simulink model "Architecture_261027_ver9"  (R2026b)
settings: Solver=FixedStepDiscrete  FixedStep=0.005
(part 2 of 2)

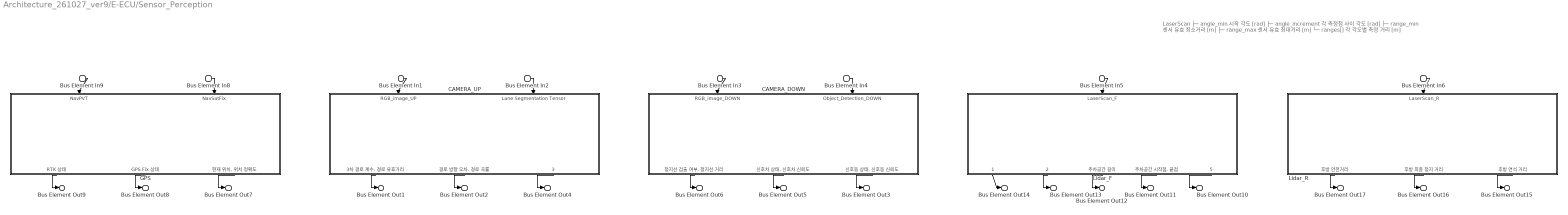
== system Architecture_261027_ver9/E-ECU/Sensor_Perception ==
  note: LaserScan
      | ├─ angle_min 시작 각도 [rad]
      | ├─ angle_increment 각 측정점 사이 각도 [rad]
      | ├─ range_min 센서 유효 최소거리 [m]
      | ├─ range_max 센서 유효 최대거리 [m]
      | └─ ranges[] 각 각도별 측정 거리 [m]
  Bus Element In1 : Inport  PortName=RGB_image_UP
  Bus Element In2 : Inport  Port=2  PortName=Lane Segmentation Tensor
  Bus Element In3 : Inport  Port=3  PortName=RGB_image_DOWN
  Bus Element In4 : Inport  Port=4  PortName=Object_Detection_DOWN
  Bus Element In5 : Inport  Port=5  PortName=LaserScan_F
  Bus Element In6 : Inport  Port=6  PortName=LaserScan_R
  Bus Element In9 : Inport  Port=7  PortName=NavPVT
  Bus Element In8 : Inport  Port=8  PortName=NavSatFix
  CAMERA_DOWN : Subsystem
      settings: PortSchema="{\"entries\":[{\"content\":{\"headerSize\":26,\"margin\":15,\"minimumSpacing\":25,\"sides\":[{\"content\":{},\"type\":\"ConnectorPlacement.EquallySpacedRectSide\",\"uuid\":\"3db2b88d-95e2-4692-a68d-7a6617ae29da\"},{\"content\":{\"side\":\"RIGHT\"},\"type\":\"ConnectorPlacement.EquallySpacedRectSide\",\"uuid\":\"d7a2bc47-76ea-49a7-91d2-0b0182d23db2\"},{\"content\":{\"connectorIds\":[\"In1\",\"In2\"],\"side\":\"TOP\"},\"type\":\"ConnectorPlacement.EquallySpacedRectSide\",\"uuid\":\"f0af930f-0cf6-4b9c-8a26-23e4e388c29c\"},{\"content\":{\"connectorIds\":[\"Out1\",\"Out2\",\"Out3\"],\"side\":\"BOTTOM\"},\"type\":\"ConnectorPlacement.EquallySpacedRectSide\",\"uuid\":\"67596a2e-158a-411e-8daf-83dd5bf86ad3\"}]},\"type\":\"ConnectorPlacement.EquallySpacedConnector\",\"uuid\":\"d65d877a-ca9e-4f5a-ba0a-bbaf7f04c4f0\"}],\"packageUris\":[\"http://schema.mathworks.com/mf0/Connector/R2020b\"],\"version\":\"1.0\"}"
  CAMERA_UP : Subsystem
      settings: PortSchema="{\"entries\":[{\"content\":{\"headerSize\":26,\"margin\":15,\"minimumSpacing\":25,\"sides\":[{\"content\":{},\"type\":\"ConnectorPlacement.EquallySpacedRectSide\",\"uuid\":\"3db2b88d-95e2-4692-a68d-7a6617ae29da\"},{\"content\":{\"side\":\"RIGHT\"},\"type\":\"ConnectorPlacement.EquallySpacedRectSide\",\"uuid\":\"d7a2bc47-76ea-49a7-91d2-0b0182d23db2\"},{\"content\":{\"connectorIds\":[\"In1\",\"In2\"],\"side\":\"TOP\"},\"type\":\"ConnectorPlacement.EquallySpacedRectSide\",\"uuid\":\"f0af930f-0cf6-4b9c-8a26-23e4e388c29c\"},{\"content\":{\"connectorIds\":[\"Out1\",\"Out2\",\"Out3\"],\"side\":\"BOTTOM\"},\"type\":\"ConnectorPlacement.EquallySpacedRectSide\",\"uuid\":\"de9f83c0-76b7-4878-914e-e95a158d2e20\"}]},\"type\":\"ConnectorPlacement.EquallySpacedConnector\",\"uuid\":\"d65d877a-ca9e-4f5a-ba0a-bbaf7f04c4f0\"}],\"packageUris\":[\"http://schema.mathworks.com/mf0/Connector/R2020b\"],\"version\":\"1.0\"}"
  GPS : Subsystem
      settings: PortSchema="{\"entries\":[{\"content\":{\"headerSize\":26,\"margin\":15,\"minimumSpacing\":25,\"sides\":[{\"content\":{},\"type\":\"ConnectorPlacement.EquallySpacedRectSide\",\"uuid\":\"3db2b88d-95e2-4692-a68d-7a6617ae29da\"},{\"content\":{\"side\":\"RIGHT\"},\"type\":\"ConnectorPlacement.EquallySpacedRectSide\",\"uuid\":\"d7a2bc47-76ea-49a7-91d2-0b0182d23db2\"},{\"content\":{\"connectorIds\":[\"In2\",\"In1\"],\"side\":\"TOP\"},\"type\":\"ConnectorPlacement.EquallySpacedRectSide\",\"uuid\":\"f0af930f-0cf6-4b9c-8a26-23e4e388c29c\"},{\"content\":{\"connectorIds\":[\"Out1\",\"Out2\",\"Out3\"],\"side\":\"BOTTOM\"},\"type\":\"ConnectorPlacement.EquallySpacedRectSide\",\"uuid\":\"c8f4bbcc-ac0b-4106-aebd-72f0ecd21f1b\"}]},\"type\":\"ConnectorPlacement.EquallySpacedConnector\",\"uuid\":\"d65d877a-ca9e-4f5a-ba0a-bbaf7f04c4f0\"}],\"packageUris\":[\"http://schema.mathworks.com/mf0/Connector/R2020b\"],\"version\":\"1.0\"}"
  Lidar_F : Subsystem
      settings: PortSchema="{\"entries\":[{\"content\":{\"headerSize\":26,\"margin\":15,\"minimumSpacing\":25,\"sides\":[{\"content\":{},\"type\":\"ConnectorPlacement.EquallySpacedRectSide\",\"uuid\":\"3db2b88d-95e2-4692-a68d-7a6617ae29da\"},{\"content\":{\"side\":\"RIGHT\"},\"type\":\"ConnectorPlacement.EquallySpacedRectSide\",\"uuid\":\"d7a2bc47-76ea-49a7-91d2-0b0182d23db2\"},{\"content\":{\"connectorIds\":[\"In1\"],\"side\":\"TOP\"},\"type\":\"ConnectorPlacement.EquallySpacedRectSide\",\"uuid\":\"f0af930f-0cf6-4b9c-8a26-23e4e388c29c\"},{\"content\":{\"connectorIds\":[\"Out1\",\"Out2\",\"Out3\",\"Out4\",\"Out5\"],\"side\":\"BOTTOM\"},\"type\":\"ConnectorPlacement.EquallySpacedRectSide\",\"uuid\":\"cd59c8ad-aa31-4ab1-b799-627b51476627\"}]},\"type\":\"ConnectorPlacement.EquallySpacedConnector\",\"uuid\":\"d65d877a-ca9e-4f5a-ba0a-bbaf7f04c4f0\"}],\"packageUris\":[\"http://schema.mathworks.com/mf0/Connector/R2020b\"],\"version\":\"1.0\"}"
  Lidar_R : Subsystem
      settings: PortSchema="{\"entries\":[{\"content\":{\"headerSize\":26,\"margin\":15,\"minimumSpacing\":25,\"sides\":[{\"content\":{},\"type\":\"ConnectorPlacement.EquallySpacedRectSide\",\"uuid\":\"3db2b88d-95e2-4692-a68d-7a6617ae29da\"},{\"content\":{\"side\":\"RIGHT\"},\"type\":\"ConnectorPlacement.EquallySpacedRectSide\",\"uuid\":\"d7a2bc47-76ea-49a7-91d2-0b0182d23db2\"},{\"content\":{\"connectorIds\":[\"In1\"],\"side\":\"TOP\"},\"type\":\"ConnectorPlacement.EquallySpacedRectSide\",\"uuid\":\"f0af930f-0cf6-4b9c-8a26-23e4e388c29c\"},{\"content\":{\"connectorIds\":[\"Out1\",\"Out2\",\"Out3\"],\"side\":\"BOTTOM\"},\"type\":\"ConnectorPlacement.EquallySpacedRectSide\",\"uuid\":\"d0e0971b-ab0f-4249-9f75-3116b1a494cb\"}]},\"type\":\"ConnectorPlacement.EquallySpacedConnector\",\"uuid\":\"d65d877a-ca9e-4f5a-ba0a-bbaf7f04c4f0\"}],\"packageUris\":[\"http://schema.mathworks.com/mf0/Connector/R2020b\"],\"version\":\"1.0\"}"
  Bus Element Out17 : Outport  PortName=후방 안전거리
  Bus Element Out16 : Outport  Port=2  PortName=후방 최종 정지 거리
  Bus Element Out15 : Outport  Port=3  PortName=후방 연석 거리
  Bus Element Out14 : Outport  Port=4  PortName=전방 주행 경로 내 장애물 여부
  Bus Element Out1 : Outport  Port=5  PortName=3차 경로 계수, 경로 유효거리
  Bus Element Out2 : Outport  Port=6  PortName=경로 방향 오차, 경로 곡률
  Bus Element Out4 : Outport  Port=7  PortName=차선/경로 유효 여부, 신뢰도, 차량 횡방향 오차
  Bus Element Out13 : Outport  Port=8  PortName=전방 장애물 거리, 폭, 좌우 위치
  Bus Element Out12 : Outport  Port=9  PortName=주차공간 길이
  Bus Element Out11 : Outport  Port=10  PortName=주차공간 시작점, 끝점
  Bus Element Out10 : Outport  Port=11  PortName=전방 연석 검출 여부, 측면 연석 거리
  Bus Element Out9 : Outport  Port=12  PortName=RTK 상태
  Bus Element Out8 : Outport  Port=13  PortName=GPS Fix 상태
  Bus Element Out5 : Outport  Port=14  PortName=신호차 상태, 신호차 신뢰도
  Bus Element Out7 : Outport  Port=15  PortName=현재 위치, 위치 정확도
  Bus Element Out6 : Outport  Port=16  PortName=정지선 검출 여부, 정지선 거리
  Bus Element Out3 : Outport  Port=17  PortName=신호등 상태, 신호등 신뢰도
  wires:
  CAMERA_DOWN/2("신호차 상태, 신호차 신뢰도") -> Bus Element Out5/1
  CAMERA_DOWN/1("정지선 검출 여부, 정지선 거리") -> Bus Element Out6/1
  CAMERA_DOWN/3("신호등 상태, 신호등 신뢰도") -> Bus Element Out3/1
  GPS/1(RTK 상태) -> Bus Element Out9/1
  GPS/2(GPS Fix 상태) -> Bus Element Out8/1
  GPS/3("현재 위치, 위치 정확도") -> Bus Element Out7/1
  Lidar_F/1(전방 주행 경로 내 장애물 여부) -> Bus Element Out14/1
  Lidar_F/2("전방 장애물 거리, 폭, 좌우 위치") -> Bus Element Out13/1
  Lidar_F/3(주차공간 길이) -> Bus Element Out12/1
  Lidar_F/4("주차공간 시작점, 끝점") -> Bus Element Out11/1
  Lidar_F/5("전방 연석 검출 여부, 측면 연석 거리") -> Bus Element Out10/1
  Lidar_R/3(후방 연석 거리) -> Bus Element Out15/1
  Lidar_R/2(후방 최종 정지 거리) -> Bus Element Out16/1
  Lidar_R/1(후방 안전거리) -> Bus Element Out17/1
  Bus Element In8/1 -> GPS/1("NavSatFix ")
  Bus Element In9/1 -> GPS/2(NavPVT)
  Bus Element In1/1 -> CAMERA_UP/1(RGB_image_UP)
  Bus Element In3/1 -> CAMERA_DOWN/1(RGB_image_DOWN)
  Bus Element In4/1 -> CAMERA_DOWN/2(Object_Detection_DOWN)
  Bus Element In6/1 -> Lidar_R/1(LaserScan_R)
  Bus Element In5/1 -> Lidar_F/1(LaserScan_F)
  Bus Element In2/1 -> CAMERA_UP/2(Lane Segmentation Tensor)
  CAMERA_UP/1("3차 경로 계수, 경로 유효거리") -> Bus Element Out1/1
  CAMERA_UP/2("경로 방향 오차, 경로 곡률") -> Bus Element Out2/1
  CAMERA_UP/3("차선/경로 유효 여부, 신뢰도, 차량 횡방향 오차") -> Bus Element Out4/1

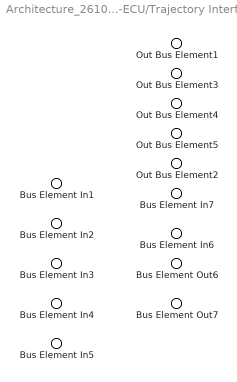
== system Architecture_261027_ver9/E-ECU/Trajectory Interface ==
  Bus Element In1 : Inport  PortName=GPS_Trajectory
  Bus Element In2 : Inport  Port=2  PortName=TParking_Trajectory
  Bus Element In3 : Inport  Port=3  PortName=ParallelParking_Trajectory
  Bus Element In4 : Inport  Port=4  PortName=Avoidance_Trajectory
  Bus Element In5 : Inport  Port=5  PortName=Camera_Trajectory
  Bus Element In7 : Inport  Port=6  PortName=Traffic_Stop_Request
  Bus Element In6 : Inport  Port=7  PortName=MRM_Stop_Request
  Out Bus Element1 : Outport  PortName=""
  Out Bus Element2 : Outport  Port=2  PortName=""
  Out Bus Element3 : Outport  Port=3  PortName=""
  Out Bus Element4 : Outport  Port=4  PortName=""
  Out Bus Element5 : Outport  Port=5  PortName=""
  Bus Element Out6 : Outport  Port=6  PortName=""
  Bus Element Out7 : Outport  Port=7  PortName=""

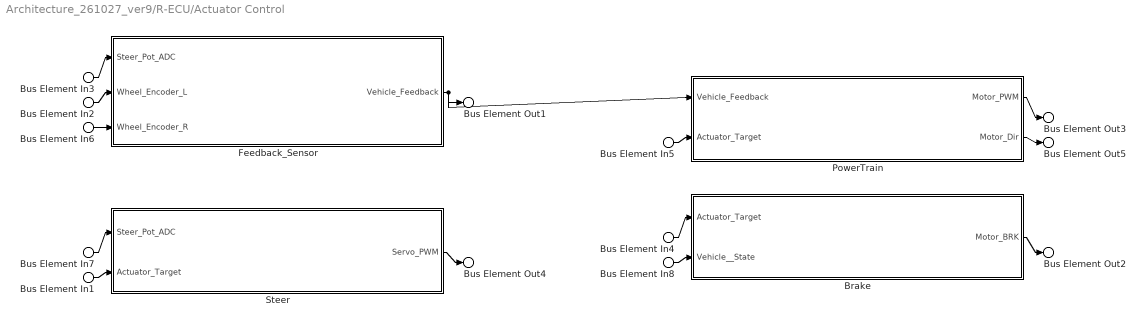
== system Architecture_261027_ver9/R-ECU/Actuator Control ==
  Bus Element In1 : Inport  PortName=Actuator_Target
  Bus Element In4 : Inport  PortName=Actuator_Target
  Bus Element In5 : Inport  PortName=Actuator_Target
  Bus Element In8 : Inport  Port=2  PortName=Vehicle__State
  Bus Element In2 : Inport  Port=3  PortName=Wheel_Encoder_L
  Bus Element In6 : Inport  Port=4  PortName=Wheel_Encoder_R
  Bus Element In3 : Inport  Port=5  PortName=Steer_Pot_ADC
  Bus Element In7 : Inport  Port=5  PortName=Steer_Pot_ADC
  Brake : Subsystem
      settings: PortSchema="{\"entries\":[{\"content\":{\"headerSize\":26,\"margin\":15,\"minimumSpacing\":25,\"sides\":[{\"content\":{\"connectorIds\":[\"In1\",\"In2\"]},\"type\":\"ConnectorPlacement.EquallySpacedRectSide\",\"uuid\":\"5be6b78a-1fb5-4892-a059-20486cb8da03\"},{\"content\":{\"connectorIds\":[\"Out1\"],\"side\":\"RIGHT\"},\"type\":\"ConnectorPlacement.EquallySpacedRectSide\",\"uuid\":\"6033bdc5-529e-4fd7-96df-de1a61a0c34f\"},{\"content\":{\"side\":\"TOP\"},\"type\":\"ConnectorPlacement.EquallySpacedRectSide\",\"uuid\":\"4d265f78-1951-4f58-a661-9dd8a9ad83fa\"}]},\"type\":\"ConnectorPlacement.EquallySpacedConnector\",\"uuid\":\"a5be31a5-398c-4cfa-a3f1-90989462f386\"}],\"packageUris\":[\"http://schema.mathworks.com/mf0/Connector/R2020b\"],\"version\":\"1.0\"}"
  Feedback_Sensor : Subsystem
      settings: PortSchema="{\"entries\":[{\"content\":{\"headerSize\":26,\"margin\":15,\"minimumSpacing\":25,\"sides\":[{\"content\":{\"connectorIds\":[\"In1\",\"In2\",\"In3\"]},\"type\":\"ConnectorPlacement.EquallySpacedRectSide\",\"uuid\":\"5be6b78a-1fb5-4892-a059-20486cb8da03\"},{\"content\":{\"connectorIds\":[\"Out1\"],\"side\":\"RIGHT\"},\"type\":\"ConnectorPlacement.EquallySpacedRectSide\",\"uuid\":\"6033bdc5-529e-4fd7-96df-de1a61a0c34f\"},{\"content\":{\"side\":\"TOP\"},\"type\":\"ConnectorPlacement.EquallySpacedRectSide\",\"uuid\":\"4d265f78-1951-4f58-a661-9dd8a9ad83fa\"}]},\"type\":\"ConnectorPlacement.EquallySpacedConnector\",\"uuid\":\"a5be31a5-398c-4cfa-a3f1-90989462f386\"}],\"packageUris\":[\"http://schema.mathworks.com/mf0/Connector/R2020b\"],\"version\":\"1.0\"}"
  PowerTrain : Subsystem
      settings: PortSchema="{\"entries\":[{\"content\":{\"headerSize\":26,\"margin\":15,\"minimumSpacing\":25,\"sides\":[{\"content\":{\"connectorIds\":[\"In1\",\"In2\"]},\"type\":\"ConnectorPlacement.EquallySpacedRectSide\",\"uuid\":\"5be6b78a-1fb5-4892-a059-20486cb8da03\"},{\"content\":{\"connectorIds\":[\"Out1\",\"Out2\"],\"side\":\"RIGHT\"},\"type\":\"ConnectorPlacement.EquallySpacedRectSide\",\"uuid\":\"6033bdc5-529e-4fd7-96df-de1a61a0c34f\"},{\"content\":{\"side\":\"TOP\"},\"type\":\"ConnectorPlacement.EquallySpacedRectSide\",\"uuid\":\"4d265f78-1951-4f58-a661-9dd8a9ad83fa\"}]},\"type\":\"ConnectorPlacement.EquallySpacedConnector\",\"uuid\":\"a5be31a5-398c-4cfa-a3f1-90989462f386\"}],\"packageUris\":[\"http://schema.mathworks.com/mf0/Connector/R2020b\"],\"version\":\"1.0\"}"
  Steer : Subsystem
      settings: PortSchema="{\"entries\":[{\"content\":{\"headerSize\":26,\"margin\":15,\"minimumSpacing\":25,\"sides\":[{\"content\":{\"connectorIds\":[\"In1\",\"In2\"]},\"type\":\"ConnectorPlacement.EquallySpacedRectSide\",\"uuid\":\"5be6b78a-1fb5-4892-a059-20486cb8da03\"},{\"content\":{\"connectorIds\":[\"Out1\"],\"side\":\"RIGHT\"},\"type\":\"ConnectorPlacement.EquallySpacedRectSide\",\"uuid\":\"6033bdc5-529e-4fd7-96df-de1a61a0c34f\"},{\"content\":{\"side\":\"TOP\"},\"type\":\"ConnectorPlacement.EquallySpacedRectSide\",\"uuid\":\"4d265f78-1951-4f58-a661-9dd8a9ad83fa\"}]},\"type\":\"ConnectorPlacement.EquallySpacedConnector\",\"uuid\":\"a5be31a5-398c-4cfa-a3f1-90989462f386\"}],\"packageUris\":[\"http://schema.mathworks.com/mf0/Connector/R2020b\"],\"version\":\"1.0\"}"
  Bus Element Out5 : Outport  PortName=Motor_DIR
  Bus Element Out1 : Outport  Port=2  PortName=Vehicle_Feedback
  Bus Element Out4 : Outport  Port=3  PortName=Servo_PWM
  Bus Element Out3 : Outport  Port=4  PortName=Motor_PWM
  Bus Element Out2 : Outport  Port=5  PortName=Motor_BRK
  wires:
  Bus Element In2/1 -> Feedback_Sensor/2(Wheel_Encoder_L)
  Bus Element In3/1 -> Feedback_Sensor/1(Steer_Pot_ADC)
  Bus Element In1/1 -> Steer/2(Actuator_Target)
  Bus Element In4/1 -> Brake/1(Actuator_Target)
  Bus Element In5/1 -> PowerTrain/2(Actuator_Target)
  Steer/1(Servo_PWM) -> Bus Element Out4/1
  Brake/1(Motor_BRK) -> Bus Element Out2/1
  PowerTrain/1(Motor_PWM) -> Bus Element Out3/1
  Feedback_Sensor/1(Vehicle_Feedback) -> PowerTrain/1(Vehicle_Feedback), Bus Element Out1/1
  PowerTrain/2(Motor_Dir) -> Bus Element Out5/1
  Bus Element In6/1 -> Feedback_Sensor/3(Wheel_Encoder_R)
  Bus Element In7/1 -> Steer/1(Steer_Pot_ADC)
  Bus Element In8/1 -> Brake/2(Vehicle__State)

== system Architecture_261027_ver9/E-ECU/ADAS_Application/Camera_Driving_App ==
  Bus Element In2 : Inport  PortName=feedback_steering_angle_deg
  Bus Element In3 : Inport  Port=2  PortName=feedback_speed
  Bus Element In4 : Inport  Port=3  PortName=차선/경로 유효 여부, 신뢰도, 차량 횡방향 오차
  Bus Element In1 : Inport  Port=4  PortName=3차 경로 계수, 경로 유효거리
  Bus Element In5 : Inport  Port=5  PortName=경로 방향 오차, 경로 곡률
  Bus Element Out1 : Outport  PortName=Camera_Trajectory

== system Architecture_261027_ver9/E-ECU/ADAS_Application/Collision_Avoidance_App ==
  Bus Element In3 : Inport  PortName=feedback_speed
  Bus Element In4 : Inport  Port=2  PortName=feedback_steering_angle_deg
  Bus Element In1 : Inport  Port=3  PortName=전방 장애물 거리, 폭, 좌우 위치
  Bus Element In2 : Inport  Port=4  PortName=주행 경로 내 장애물 여부
  Bus Element In5 : Inport  Port=5  PortName=후방 안전거리
  Bus Element Out1 : Outport  PortName=Avoidance_Trajectory

== system Architecture_261027_ver9/E-ECU/ADAS_Application/GPS_Driving_App ==
  Bus Element In5 : Inport  PortName=Lane_num
  Bus Element In3 : Inport  Port=2  PortName=feedback_speed
  Bus Element In1 : Inport  Port=3  PortName=현재 위치, 위치 정확도
  Bus Element In2 : Inport  Port=4  PortName=GPS Fix 상태
  Bus Element In6 : Inport  Port=5  PortName=RTK 상태
  Bus Element In4 : Inport  Port=6  PortName=feedback_steering_angle_deg
  Bus Element Out1 : Outport  PortName=Waypoint_Trajectory

== system Architecture_261027_ver9/E-ECU/ADAS_Application/Lane_select_App ==
  Bus Element In2 : Inport  PortName=신호차 상태, 신호차 신뢰도
  Bus Element Out1 : Outport  PortName=Lane_num

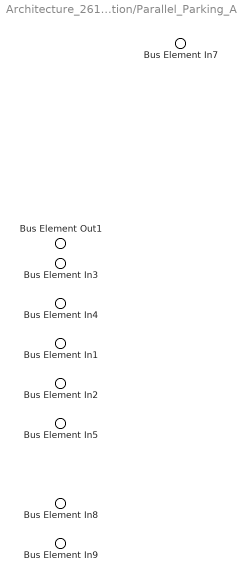
== system Architecture_261027_ver9/E-ECU/ADAS_Application/Parallel_Parking_App ==
  Bus Element In7 : Inport  PortName=후방 안전거리
  Bus Element In3 : Inport  Port=2  PortName=feedback_speed
  Bus Element In4 : Inport  Port=3  PortName=feedback_steering_angle_deg
  Bus Element In1 : Inport  Port=4  PortName=전방 연석 검출 여부, 측면 연석 거리
  Bus Element In2 : Inport  Port=5  PortName=주차공간 시작점, 끝점
  Bus Element In5 : Inport  Port=6  PortName=주차공간 길이
  Bus Element In8 : Inport  Port=7  PortName=후방 최종 정지 거리
  Bus Element In9 : Inport  Port=8  PortName=후방 연석 거리
  Bus Element Out1 : Outport  PortName=ParallelParking_Trajectory

== system Architecture_261027_ver9/E-ECU/ADAS_Application/Sudden_Stop_App ==
  Bus Element In2 : Inport  PortName=feedback_speed
  Bus Element In3 : Inport  Port=2  PortName=주행 경로 내 장애물 여부
  Bus Element Out1 : Outport  PortName=MRM_Stop_Request

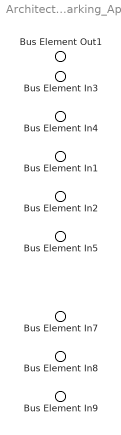
== system Architecture_261027_ver9/E-ECU/ADAS_Application/T_Parking_App ==
  Bus Element In3 : Inport  PortName=feedback_speed
  Bus Element In4 : Inport  Port=2  PortName=feedback_steering_angle_deg
  Bus Element In1 : Inport  Port=3  PortName=전방 연석 검출 여부, 측면 연석 거리
  Bus Element In2 : Inport  Port=4  PortName=주차공간 시작점, 끝점
  Bus Element In5 : Inport  Port=5  PortName=주차공간 길이
  Bus Element In7 : Inport  Port=6  PortName=후방 연석 거리
  Bus Element In8 : Inport  Port=7  PortName=후방 최종 정지 거리
  Bus Element In9 : Inport  Port=8  PortName=후방 안전거리
  Bus Element Out1 : Outport  PortName=TParking_Trajectory

== system Architecture_261027_ver9/E-ECU/ADAS_Application/Traffic_App ==
  Bus Element In2 : Inport  PortName=신호등 상태, 신호등 신뢰도
  Bus Element In3 : Inport  Port=2  PortName=정지선 검출 여부, 정지선 거리
  Bus Element In1 : Inport  Port=3  PortName=feedback_speed
  Bus Element Out1 : Outport  PortName=Traffic_Stop_Request

== system Architecture_261027_ver9/E-ECU/Sensor_Perception/CAMERA_DOWN ==
  Bus Element In1 : Inport  PortName=RGB_image_DOWN
  Bus Element In2 : Inport  Port=2  PortName=Object_Detection_DOWN
  Bus Element Out2 : Outport  PortName=정지선 검출 여부, 정지선 거리
  Bus Element Out1 : Outport  Port=2  PortName=신호차 상태, 신호차 신뢰도
  Bus Element Out3 : Outport  Port=3  PortName=신호등 상태, 신호등 신뢰도

== system Architecture_261027_ver9/E-ECU/Sensor_Perception/CAMERA_UP ==
  Bus Element In1 : Inport  PortName=RGB_image_UP
  Bus Element In2 : Inport  Port=2  PortName=Lane Segmentation Tensor
  Bus Element Out1 : Outport  PortName=3차 경로 계수, 경로 유효거리
  Bus Element Out2 : Outport  Port=2  PortName=경로 방향 오차, 경로 곡률
  Bus Element Out3 : Outport  Port=3  PortName=차선/경로 유효 여부, 신뢰도, 차량 횡방향 오차

== system Architecture_261027_ver9/E-ECU/Sensor_Perception/GPS ==
  Bus Element In1 : Inport  PortName=NavSatFix
  Bus Element In2 : Inport  Port=2  PortName=NavPVT
  Bus Element Out1 : Outport  PortName=RTK 상태
  Bus Element Out2 : Outport  Port=2  PortName=GPS Fix 상태
  Bus Element Out3 : Outport  Port=3  PortName=현재 위치, 위치 정확도

== system Architecture_261027_ver9/E-ECU/Sensor_Perception/Lidar_F ==
  Bus Element In1 : Inport  PortName=LaserScan_F
  Bus Element Out1 : Outport  PortName=전방 주행 경로 내 장애물 여부
  Bus Element Out2 : Outport  Port=2  PortName=전방 장애물 거리, 폭, 좌우 위치
  Bus Element Out3 : Outport  Port=3  PortName=주차공간 길이
  Bus Element Out4 : Outport  Port=4  PortName=주차공간 시작점, 끝점
  Bus Element Out5 : Outport  Port=5  PortName=전방 연석 검출 여부, 측면 연석 거리

== system Architecture_261027_ver9/E-ECU/Sensor_Perception/Lidar_R ==
  Bus Element In1 : Inport  PortName=LaserScan_R
  Bus Element Out3 : Outport  PortName=후방 안전거리
  Bus Element Out2 : Outport  Port=2  PortName=후방 최종 정지 거리
  Bus Element Out1 : Outport  Port=3  PortName=후방 연석 거리

== system Architecture_261027_ver9/R-ECU/Actuator Control/Brake ==
  note: Brake Condition Check: 정지·구동 비활성·안전 조건을 확인해 브레이크 작동 여부를 판단한다.
      | Brake Command: 판단된 브레이크 요청을 실제 Motor_BRK 제어 신호로 변환한다.
  Bus Element In1 : Inport  PortName=Actuator_Target
  Bus Element In2 : Inport  Port=2  PortName=Vehicle__State
  Brake : ModelReference  ModelNameDialog=Brake  SimulationMode=Normal  ModelReferenceVersion=1.8
      settings: PortSchema="{\"entries\":[{\"content\":{\"headerSize\":38,\"margin\":15,\"minimumSpacing\":25,\"sides\":[{\"content\":{},\"type\":\"ConnectorPlacement.EquallySpacedRectSide\",\"uuid\":\"3ba9c497-a723-46b8-81dd-1f7ca6a23c01\"},{\"content\":{\"side\":\"RIGHT\"},\"type\":\"ConnectorPlacement.EquallySpacedRectSide\",\"uuid\":\"d9088a6a-926e-4236-98b4-eead6aef3cee\"},{\"content\":{\"side\":\"TOP\"},\"type\":\"ConnectorPlacement.EquallySpacedRectSide\",\"uuid\":\"7a0b5e73-9353-4c95-99cb-27715f315123\"}]},\"type\":\"ConnectorPlacement.EquallySpacedConnector\",\"uuid\":\"e3d9f0ba-d452-4121-9c90-7bb8e9382a1f\"}],\"packageUris\":[\"http://schema.mathworks.com/mf0/Connector/R2020b\"],\"version\":\"1.0\"}"
  Brake Condition Check : Subsystem
      settings: PortSchema="{\"entries\":[{\"content\":{\"headerSize\":26,\"margin\":15,\"minimumSpacing\":25,\"sides\":[{\"content\":{\"connectorIds\":[\"In1\"]},\"type\":\"ConnectorPlacement.EquallySpacedRectSide\",\"uuid\":\"3db2b88d-95e2-4692-a68d-7a6617ae29da\"},{\"content\":{\"connectorIds\":[\"Out1\"],\"side\":\"RIGHT\"},\"type\":\"ConnectorPlacement.EquallySpacedRectSide\",\"uuid\":\"d7a2bc47-76ea-49a7-91d2-0b0182d23db2\"},{\"content\":{\"side\":\"TOP\"},\"type\":\"ConnectorPlacement.EquallySpacedRectSide\",\"uuid\":\"f0af930f-0cf6-4b9c-8a26-23e4e388c29c\"}]},\"type\":\"ConnectorPlacement.EquallySpacedConnector\",\"uuid\":\"d65d877a-ca9e-4f5a-ba0a-bbaf7f04c4f0\"}],\"packageUris\":[\"http://schema.mathworks.com/mf0/Connector/R2020b\"],\"version\":\"1.0\"}"
  Component : Subsystem
      settings: PortSchema="{\"entries\":[{\"content\":{\"headerSize\":26,\"margin\":15,\"minimumSpacing\":25,\"sides\":[{\"content\":{\"connectorIds\":[\"In1\"]},\"type\":\"ConnectorPlacement.EquallySpacedRectSide\",\"uuid\":\"3db2b88d-95e2-4692-a68d-7a6617ae29da\"},{\"content\":{\"connectorIds\":[\"Out1\"],\"side\":\"RIGHT\"},\"type\":\"ConnectorPlacement.EquallySpacedRectSide\",\"uuid\":\"d7a2bc47-76ea-49a7-91d2-0b0182d23db2\"},{\"content\":{\"side\":\"TOP\"},\"type\":\"ConnectorPlacement.EquallySpacedRectSide\",\"uuid\":\"f0af930f-0cf6-4b9c-8a26-23e4e388c29c\"}]},\"type\":\"ConnectorPlacement.EquallySpacedConnector\",\"uuid\":\"d65d877a-ca9e-4f5a-ba0a-bbaf7f04c4f0\"}],\"packageUris\":[\"http://schema.mathworks.com/mf0/Connector/R2020b\"],\"version\":\"1.0\"}"
  Bus Element Out1 : Outport  PortName=Motor_BRK
  wires:
  Bus Element In1/1 -> Brake Condition Check/1(Actuator_Target)
  Brake Condition Check/1(Brake_Request) -> Component/1(Brake_Request)
  Component/1(Motor_BRK) -> Bus Element Out1/1

== system Architecture_261027_ver9/R-ECU/Actuator Control/Feedback_Sensor ==
  note: Steering Feedback: 조향 포텐셔미터 ADC 값을 실제 조향각으로 변환한다.
      | Wheel Speed Feedback: 좌·우 휠 엔코더 값을 이용해 실제 차량 속도를 계산한다.
      | Feedback Valid Check: 조향각과 속도 피드백이 정상 범위이며 사용 가능한 값인지 확인한다.
      | Vehicle Feedback Build: 조향각·차속·유효 상태를 묶어 Vehicle_Feedback 으로 출력한다.
  Bus Element In1 : Inport  PortName=Steer_Pot_ADC
  Bus Element In2 : Inport  Port=2  PortName=Wheel_Encoder_L
  Bus Element In3 : Inport  Port=3  PortName=Wheel_Encoder_R
  Feedback Valid Check : Subsystem
      settings: PortSchema="{\"entries\":[{\"content\":{\"headerSize\":26,\"margin\":15,\"minimumSpacing\":25,\"sides\":[{\"content\":{\"connectorIds\":[\"In1\",\"In2\"]},\"type\":\"ConnectorPlacement.EquallySpacedRectSide\",\"uuid\":\"3db2b88d-95e2-4692-a68d-7a6617ae29da\"},{\"content\":{\"connectorIds\":[\"Out1\",\"Out2\"],\"side\":\"RIGHT\"},\"type\":\"ConnectorPlacement.EquallySpacedRectSide\",\"uuid\":\"d7a2bc47-76ea-49a7-91d2-0b0182d23db2\"},{\"content\":{\"side\":\"TOP\"},\"type\":\"ConnectorPlacement.EquallySpacedRectSide\",\"uuid\":\"f0af930f-0cf6-4b9c-8a26-23e4e388c29c\"}]},\"type\":\"ConnectorPlacement.EquallySpacedConnector\",\"uuid\":\"d65d877a-ca9e-4f5a-ba0a-bbaf7f04c4f0\"}],\"packageUris\":[\"http://schema.mathworks.com/mf0/Connector/R2020b\"],\"version\":\"1.0\"}"
  Steering Feedback : Subsystem
      settings: PortSchema="{\"entries\":[{\"content\":{\"headerSize\":26,\"margin\":15,\"minimumSpacing\":25,\"sides\":[{\"content\":{\"connectorIds\":[\"In1\"]},\"type\":\"ConnectorPlacement.EquallySpacedRectSide\",\"uuid\":\"3db2b88d-95e2-4692-a68d-7a6617ae29da\"},{\"content\":{\"connectorIds\":[\"Out1\"],\"side\":\"RIGHT\"},\"type\":\"ConnectorPlacement.EquallySpacedRectSide\",\"uuid\":\"d7a2bc47-76ea-49a7-91d2-0b0182d23db2\"},{\"content\":{\"side\":\"TOP\"},\"type\":\"ConnectorPlacement.EquallySpacedRectSide\",\"uuid\":\"f0af930f-0cf6-4b9c-8a26-23e4e388c29c\"}]},\"type\":\"ConnectorPlacement.EquallySpacedConnector\",\"uuid\":\"d65d877a-ca9e-4f5a-ba0a-bbaf7f04c4f0\"}],\"packageUris\":[\"http://schema.mathworks.com/mf0/Connector/R2020b\"],\"version\":\"1.0\"}"
  Vehicle Feedback Build : Subsystem
      settings: PortSchema="{\"entries\":[{\"content\":{\"headerSize\":26,\"margin\":15,\"minimumSpacing\":25,\"sides\":[{\"content\":{\"connectorIds\":[\"In1\",\"In2\",\"In3\",\"In4\"]},\"type\":\"ConnectorPlacement.EquallySpacedRectSide\",\"uuid\":\"3db2b88d-95e2-4692-a68d-7a6617ae29da\"},{\"content\":{\"connectorIds\":[\"Out1\"],\"side\":\"RIGHT\"},\"type\":\"ConnectorPlacement.EquallySpacedRectSide\",\"uuid\":\"d7a2bc47-76ea-49a7-91d2-0b0182d23db2\"},{\"content\":{\"side\":\"TOP\"},\"type\":\"ConnectorPlacement.EquallySpacedRectSide\",\"uuid\":\"f0af930f-0cf6-4b9c-8a26-23e4e388c29c\"}]},\"type\":\"ConnectorPlacement.EquallySpacedConnector\",\"uuid\":\"d65d877a-ca9e-4f5a-ba0a-bbaf7f04c4f0\"}],\"packageUris\":[\"http://schema.mathworks.com/mf0/Connector/R2020b\"],\"version\":\"1.0\"}"
  Wheel Speed Feedback : Subsystem
      settings: PortSchema="{\"entries\":[{\"content\":{\"headerSize\":26,\"margin\":15,\"minimumSpacing\":25,\"sides\":[{\"content\":{\"connectorIds\":[\"In1\",\"In2\"]},\"type\":\"ConnectorPlacement.EquallySpacedRectSide\",\"uuid\":\"3db2b88d-95e2-4692-a68d-7a6617ae29da\"},{\"content\":{\"connectorIds\":[\"Out1\"],\"side\":\"RIGHT\"},\"type\":\"ConnectorPlacement.EquallySpacedRectSide\",\"uuid\":\"d7a2bc47-76ea-49a7-91d2-0b0182d23db2\"},{\"content\":{\"side\":\"TOP\"},\"type\":\"ConnectorPlacement.EquallySpacedRectSide\",\"uuid\":\"f0af930f-0cf6-4b9c-8a26-23e4e388c29c\"}]},\"type\":\"ConnectorPlacement.EquallySpacedConnector\",\"uuid\":\"d65d877a-ca9e-4f5a-ba0a-bbaf7f04c4f0\"}],\"packageUris\":[\"http://schema.mathworks.com/mf0/Connector/R2020b\"],\"version\":\"1.0\"}"
  feedback sensor : ModelReference  ModelNameDialog=feedbackSensor  SimulationMode=Normal  ModelReferenceVersion=1.8
      settings: PortSchema="{\"entries\":[{\"content\":{\"headerSize\":38,\"margin\":15,\"minimumSpacing\":25,\"sides\":[{\"content\":{},\"type\":\"ConnectorPlacement.EquallySpacedRectSide\",\"uuid\":\"3ba9c497-a723-46b8-81dd-1f7ca6a23c01\"},{\"content\":{\"side\":\"RIGHT\"},\"type\":\"ConnectorPlacement.EquallySpacedRectSide\",\"uuid\":\"d9088a6a-926e-4236-98b4-eead6aef3cee\"},{\"content\":{\"side\":\"TOP\"},\"type\":\"ConnectorPlacement.EquallySpacedRectSide\",\"uuid\":\"7a0b5e73-9353-4c95-99cb-27715f315123\"}]},\"type\":\"ConnectorPlacement.EquallySpacedConnector\",\"uuid\":\"e3d9f0ba-d452-4121-9c90-7bb8e9382a1f\"}],\"packageUris\":[\"http://schema.mathworks.com/mf0/Connector/R2020b\"],\"version\":\"1.0\"}"
  Bus Element Out1 : Outport  PortName=Vehicle_Feedback
  wires:
  Bus Element In1/1 -> Steering Feedback/1(Steer_Pot_ADC)
  Bus Element In2/1 -> Wheel Speed Feedback/1(Wheel_Encoder_L)
  Bus Element In3/1 -> Wheel Speed Feedback/2(Wheel_Encoder_R)
  Steering Feedback/1(Measured_Steering) -> Vehicle Feedback Build/1(Measured_Steering), Feedback Valid Check/1(Measured_Steering)
  Wheel Speed Feedback/1(Measured_Speed) -> Vehicle Feedback Build/4(Measured_Speed), Feedback Valid Check/2(Measured_Speed)
  Feedback Valid Check/1(Steering_Valid) -> Vehicle Feedback Build/2(Steering_Valid)
  Feedback Valid Check/2(Speed_Valid) -> Vehicle Feedback Build/3(Speed_Valid)
  Vehicle Feedback Build/1(Vehicle_Feedback) -> Bus Element Out1/1

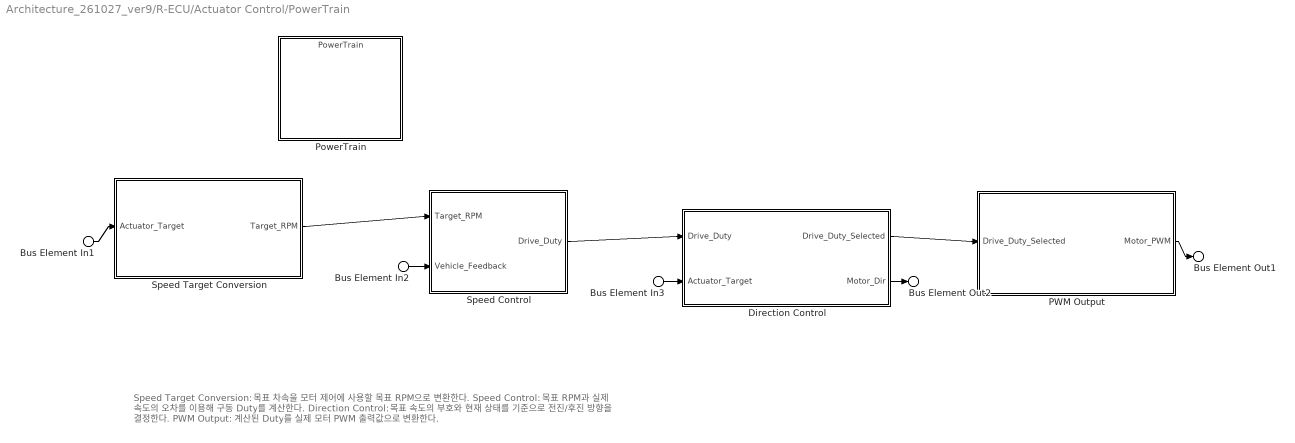
== system Architecture_261027_ver9/R-ECU/Actuator Control/PowerTrain ==
  note: Speed Target Conversion: 목표 차속을 모터 제어에 사용할 목표 RPM으로 변환한다.
      | Speed Control: 목표 RPM과 실제 속도의 오차를 이용해 구동 Duty를 계산한다.
      | Direction Control: 목표 속도의 부호와 현재 상태를 기준으로 전진/후진 방향을 결정한다.
      | PWM Output: 계산된 Duty를 실제 모터 PWM 출력값으로 변환한다.
  Bus Element In2 : Inport  PortName=Vehicle_Feedback
  Bus Element In1 : Inport  Port=2  PortName=Actuator_Target
  Bus Element In3 : Inport  Port=2  PortName=Actuator_Target
  Direction Control : Subsystem
      settings: PortSchema="{\"entries\":[{\"content\":{\"headerSize\":26,\"margin\":15,\"minimumSpacing\":25,\"sides\":[{\"content\":{\"connectorIds\":[\"In1\",\"In2\"]},\"type\":\"ConnectorPlacement.EquallySpacedRectSide\",\"uuid\":\"3db2b88d-95e2-4692-a68d-7a6617ae29da\"},{\"content\":{\"connectorIds\":[\"Out1\",\"Out2\"],\"side\":\"RIGHT\"},\"type\":\"ConnectorPlacement.EquallySpacedRectSide\",\"uuid\":\"d7a2bc47-76ea-49a7-91d2-0b0182d23db2\"},{\"content\":{\"side\":\"TOP\"},\"type\":\"ConnectorPlacement.EquallySpacedRectSide\",\"uuid\":\"f0af930f-0cf6-4b9c-8a26-23e4e388c29c\"}]},\"type\":\"ConnectorPlacement.EquallySpacedConnector\",\"uuid\":\"d65d877a-ca9e-4f5a-ba0a-bbaf7f04c4f0\"}],\"packageUris\":[\"http://schema.mathworks.com/mf0/Connector/R2020b\"],\"version\":\"1.0\"}"
  PWM Output : Subsystem
      settings: PortSchema="{\"entries\":[{\"content\":{\"headerSize\":26,\"margin\":15,\"minimumSpacing\":25,\"sides\":[{\"content\":{\"connectorIds\":[\"In1\"]},\"type\":\"ConnectorPlacement.EquallySpacedRectSide\",\"uuid\":\"3db2b88d-95e2-4692-a68d-7a6617ae29da\"},{\"content\":{\"connectorIds\":[\"Out1\"],\"side\":\"RIGHT\"},\"type\":\"ConnectorPlacement.EquallySpacedRectSide\",\"uuid\":\"d7a2bc47-76ea-49a7-91d2-0b0182d23db2\"},{\"content\":{\"side\":\"TOP\"},\"type\":\"ConnectorPlacement.EquallySpacedRectSide\",\"uuid\":\"f0af930f-0cf6-4b9c-8a26-23e4e388c29c\"}]},\"type\":\"ConnectorPlacement.EquallySpacedConnector\",\"uuid\":\"d65d877a-ca9e-4f5a-ba0a-bbaf7f04c4f0\"}],\"packageUris\":[\"http://schema.mathworks.com/mf0/Connector/R2020b\"],\"version\":\"1.0\"}"
  PowerTrain : ModelReference  ModelNameDialog=PowerTrain  SimulationMode=Normal  ModelReferenceVersion=1.8
      settings: PortSchema="{\"entries\":[{\"content\":{\"headerSize\":38,\"margin\":15,\"minimumSpacing\":25,\"sides\":[{\"content\":{},\"type\":\"ConnectorPlacement.EquallySpacedRectSide\",\"uuid\":\"3ba9c497-a723-46b8-81dd-1f7ca6a23c01\"},{\"content\":{\"side\":\"RIGHT\"},\"type\":\"ConnectorPlacement.EquallySpacedRectSide\",\"uuid\":\"d9088a6a-926e-4236-98b4-eead6aef3cee\"},{\"content\":{\"side\":\"TOP\"},\"type\":\"ConnectorPlacement.EquallySpacedRectSide\",\"uuid\":\"7a0b5e73-9353-4c95-99cb-27715f315123\"}]},\"type\":\"ConnectorPlacement.EquallySpacedConnector\",\"uuid\":\"e3d9f0ba-d452-4121-9c90-7bb8e9382a1f\"}],\"packageUris\":[\"http://schema.mathworks.com/mf0/Connector/R2020b\"],\"version\":\"1.0\"}"
  Speed Control : Subsystem
      settings: PortSchema="{\"entries\":[{\"content\":{\"headerSize\":26,\"margin\":15,\"minimumSpacing\":25,\"sides\":[{\"content\":{\"connectorIds\":[\"In1\",\"In2\"]},\"type\":\"ConnectorPlacement.EquallySpacedRectSide\",\"uuid\":\"3db2b88d-95e2-4692-a68d-7a6617ae29da\"},{\"content\":{\"connectorIds\":[\"Out1\"],\"side\":\"RIGHT\"},\"type\":\"ConnectorPlacement.EquallySpacedRectSide\",\"uuid\":\"d7a2bc47-76ea-49a7-91d2-0b0182d23db2\"},{\"content\":{\"side\":\"TOP\"},\"type\":\"ConnectorPlacement.EquallySpacedRectSide\",\"uuid\":\"f0af930f-0cf6-4b9c-8a26-23e4e388c29c\"}]},\"type\":\"ConnectorPlacement.EquallySpacedConnector\",\"uuid\":\"d65d877a-ca9e-4f5a-ba0a-bbaf7f04c4f0\"}],\"packageUris\":[\"http://schema.mathworks.com/mf0/Connector/R2020b\"],\"version\":\"1.0\"}"
  Speed Target Conversion : Subsystem
      settings: PortSchema="{\"entries\":[{\"content\":{\"headerSize\":26,\"margin\":15,\"minimumSpacing\":25,\"sides\":[{\"content\":{\"connectorIds\":[\"In1\"]},\"type\":\"ConnectorPlacement.EquallySpacedRectSide\",\"uuid\":\"3db2b88d-95e2-4692-a68d-7a6617ae29da\"},{\"content\":{\"connectorIds\":[\"Out1\"],\"side\":\"RIGHT\"},\"type\":\"ConnectorPlacement.EquallySpacedRectSide\",\"uuid\":\"d7a2bc47-76ea-49a7-91d2-0b0182d23db2\"},{\"content\":{\"side\":\"TOP\"},\"type\":\"ConnectorPlacement.EquallySpacedRectSide\",\"uuid\":\"f0af930f-0cf6-4b9c-8a26-23e4e388c29c\"},{\"content\":{\"side\":\"BOTTOM\"},\"type\":\"ConnectorPlacement.EquallySpacedRectSide\",\"uuid\":\"c986c54c-f31a-4486-8200-a29956ab34db\"}]},\"type\":\"ConnectorPlacement.EquallySpacedConnector\",\"uuid\":\"d65d877a-ca9e-4f5a-ba0a-bbaf7f04c4f0\"}],\"packageUris\":[\"http://schema.mathworks.com/mf0/Connector/R2020b\"],\"version\":\"1.0\"}"
  Bus Element Out1 : Outport  PortName=Motor_PWM
  Bus Element Out2 : Outport  Port=2  PortName=Motor_Dir
  wires:
  Bus Element In1/1 -> Speed Target Conversion/1(Actuator_Target)
  Speed Target Conversion/1(Target_RPM) -> Speed Control/1(Target_RPM)
  Bus Element In2/1 -> Speed Control/2(Vehicle_Feedback)
  Speed Control/1(Drive_Duty) -> Direction Control/1(Drive_Duty)
  Bus Element In3/1 -> Direction Control/2(Actuator_Target)
  Direction Control/1(Drive_Duty_Selected) -> PWM Output/1(Drive_Duty_Selected)
  PWM Output/1(Motor_PWM) -> Bus Element Out1/1
  Direction Control/2(Motor_Dir) -> Bus Element Out2/1

== system Architecture_261027_ver9/R-ECU/Actuator Control/Steer ==
  note: 1. Steering Target Conversion
      | 기능: 목표 조향각을 조향 포텐셔미터 기준의 목표 ADC 값으로 변환한다.
      | 2. Steering Error Calculation
      | 기능: 목표 ADC와 현재 조향 ADC의 차이를 계산한다.
      | 3. Steering Control
      | 기능: 조향 오차를 이용해 PID 제어값을 계산한다.
      | 4. Servo PWM Output
      | 기능: PID 결과를 제한·보정한 뒤 실제 서보 PWM 신호로 출력한다.
  Bus Element In2 : Inport  PortName=Steer_Pot_ADC
  Bus Element In1 : Inport  Port=2  PortName=Actuator_Target
  Servo PWM Output : Subsystem
      settings: PortSchema="{\"entries\":[{\"content\":{\"headerSize\":26,\"margin\":15,\"minimumSpacing\":25,\"sides\":[{\"content\":{\"connectorIds\":[\"In1\"]},\"type\":\"ConnectorPlacement.EquallySpacedRectSide\",\"uuid\":\"3db2b88d-95e2-4692-a68d-7a6617ae29da\"},{\"content\":{\"connectorIds\":[\"Out1\"],\"side\":\"RIGHT\"},\"type\":\"ConnectorPlacement.EquallySpacedRectSide\",\"uuid\":\"d7a2bc47-76ea-49a7-91d2-0b0182d23db2\"},{\"content\":{\"side\":\"TOP\"},\"type\":\"ConnectorPlacement.EquallySpacedRectSide\",\"uuid\":\"f0af930f-0cf6-4b9c-8a26-23e4e388c29c\"}]},\"type\":\"ConnectorPlacement.EquallySpacedConnector\",\"uuid\":\"d65d877a-ca9e-4f5a-ba0a-bbaf7f04c4f0\"}],\"packageUris\":[\"http://schema.mathworks.com/mf0/Connector/R2020b\"],\"version\":\"1.0\"}"
  Steering Control : Subsystem
      settings: PortSchema="{\"entries\":[{\"content\":{\"headerSize\":26,\"margin\":15,\"minimumSpacing\":25,\"sides\":[{\"content\":{\"connectorIds\":[\"In1\"]},\"type\":\"ConnectorPlacement.EquallySpacedRectSide\",\"uuid\":\"3db2b88d-95e2-4692-a68d-7a6617ae29da\"},{\"content\":{\"connectorIds\":[\"Out1\"],\"side\":\"RIGHT\"},\"type\":\"ConnectorPlacement.EquallySpacedRectSide\",\"uuid\":\"d7a2bc47-76ea-49a7-91d2-0b0182d23db2\"},{\"content\":{\"side\":\"TOP\"},\"type\":\"ConnectorPlacement.EquallySpacedRectSide\",\"uuid\":\"f0af930f-0cf6-4b9c-8a26-23e4e388c29c\"}]},\"type\":\"ConnectorPlacement.EquallySpacedConnector\",\"uuid\":\"d65d877a-ca9e-4f5a-ba0a-bbaf7f04c4f0\"}],\"packageUris\":[\"http://schema.mathworks.com/mf0/Connector/R2020b\"],\"version\":\"1.0\"}"
  Steering Error Calculation : Subsystem
      settings: PortSchema="{\"entries\":[{\"content\":{\"headerSize\":26,\"margin\":15,\"minimumSpacing\":25,\"sides\":[{\"content\":{\"connectorIds\":[\"In1\",\"In2\"]},\"type\":\"ConnectorPlacement.EquallySpacedRectSide\",\"uuid\":\"3db2b88d-95e2-4692-a68d-7a6617ae29da\"},{\"content\":{\"connectorIds\":[\"Out1\"],\"side\":\"RIGHT\"},\"type\":\"ConnectorPlacement.EquallySpacedRectSide\",\"uuid\":\"d7a2bc47-76ea-49a7-91d2-0b0182d23db2\"},{\"content\":{\"side\":\"TOP\"},\"type\":\"ConnectorPlacement.EquallySpacedRectSide\",\"uuid\":\"f0af930f-0cf6-4b9c-8a26-23e4e388c29c\"}]},\"type\":\"ConnectorPlacement.EquallySpacedConnector\",\"uuid\":\"d65d877a-ca9e-4f5a-ba0a-bbaf7f04c4f0\"}],\"packageUris\":[\"http://schema.mathworks.com/mf0/Connector/R2020b\"],\"version\":\"1.0\"}"
  Steering Target Conversion : Subsystem
      settings: PortSchema="{\"entries\":[{\"content\":{\"headerSize\":26,\"margin\":15,\"minimumSpacing\":25,\"sides\":[{\"content\":{\"connectorIds\":[\"In1\"]},\"type\":\"ConnectorPlacement.EquallySpacedRectSide\",\"uuid\":\"3db2b88d-95e2-4692-a68d-7a6617ae29da\"},{\"content\":{\"connectorIds\":[\"Out1\"],\"side\":\"RIGHT\"},\"type\":\"ConnectorPlacement.EquallySpacedRectSide\",\"uuid\":\"d7a2bc47-76ea-49a7-91d2-0b0182d23db2\"},{\"content\":{\"side\":\"TOP\"},\"type\":\"ConnectorPlacement.EquallySpacedRectSide\",\"uuid\":\"f0af930f-0cf6-4b9c-8a26-23e4e388c29c\"}]},\"type\":\"ConnectorPlacement.EquallySpacedConnector\",\"uuid\":\"d65d877a-ca9e-4f5a-ba0a-bbaf7f04c4f0\"}],\"packageUris\":[\"http://schema.mathworks.com/mf0/Connector/R2020b\"],\"version\":\"1.0\"}"
  steer : ModelReference  ModelNameDialog=steer  SimulationMode=Normal  ModelReferenceVersion=1.8
      settings: PortSchema="{\"entries\":[{\"content\":{\"headerSize\":38,\"margin\":15,\"minimumSpacing\":25,\"sides\":[{\"content\":{},\"type\":\"ConnectorPlacement.EquallySpacedRectSide\",\"uuid\":\"3ba9c497-a723-46b8-81dd-1f7ca6a23c01\"},{\"content\":{\"side\":\"RIGHT\"},\"type\":\"ConnectorPlacement.EquallySpacedRectSide\",\"uuid\":\"d9088a6a-926e-4236-98b4-eead6aef3cee\"},{\"content\":{\"side\":\"TOP\"},\"type\":\"ConnectorPlacement.EquallySpacedRectSide\",\"uuid\":\"7a0b5e73-9353-4c95-99cb-27715f315123\"}]},\"type\":\"ConnectorPlacement.EquallySpacedConnector\",\"uuid\":\"e3d9f0ba-d452-4121-9c90-7bb8e9382a1f\"}],\"packageUris\":[\"http://schema.mathworks.com/mf0/Connector/R2020b\"],\"version\":\"1.0\"}"
  Bus Element Out1 : Outport  PortName=Servo_PWM
  wires:
  Bus Element In1/1 -> Steering Target Conversion/1(Actuator_Target)
  Steering Target Conversion/1(Target_Steering_ADC) -> Steering Error Calculation/1(Target_Steering_ADC)
  Bus Element In2/1 -> Steering Error Calculation/2(Steer_Pot_ADC)
  Steering Error Calculation/1(Steering_Error) -> Steering Control/1(Steering_Error)
  Steering Control/1(Steering_Control_Output) -> Servo PWM Output/1(Steering_Control_Output)
  Servo PWM Output/1(Servo_PWM) -> Bus Element Out1/1

== system Architecture_261027_ver9/R-ECU/Actuator Control/Brake/Brake Condition Check ==
  Bus Element In1 : Inport  PortName=Actuator_Target
  Bus Element Out1 : Outport  PortName=Brake_Request

== system Architecture_261027_ver9/R-ECU/Actuator Control/Brake/Component ==
  Bus Element In1 : Inport  PortName=Brake_Request
  Bus Element Out1 : Outport  PortName=Motor_BRK

== system Architecture_261027_ver9/R-ECU/Actuator Control/Feedback_Sensor/Feedback Valid Check ==
  Bus Element In1 : Inport  PortName=Measured_Steering
  Bus Element In2 : Inport  Port=2  PortName=Measured_Speed
  Bus Element Out1 : Outport  PortName=Steering_Valid
  Bus Element Out2 : Outport  Port=2  PortName=Speed_Valid

== system Architecture_261027_ver9/R-ECU/Actuator Control/Feedback_Sensor/Steering Feedback ==
  Bus Element In1 : Inport  PortName=Steer_Pot_ADC
  Bus Element Out1 : Outport  PortName=Measured_Steering

== system Architecture_261027_ver9/R-ECU/Actuator Control/Feedback_Sensor/Vehicle Feedback Build ==
  Bus Element In3 : Inport  PortName=Measured_Steering
  Bus Element In1 : Inport  Port=2  PortName=Steering_Valid
  Bus Element In2 : Inport  Port=3  PortName=Speed_Valid
  Bus Element In4 : Inport  Port=4  PortName=Measured_Speed
  Bus Element Out1 : Outport  PortName=Vehicle_Feedback

== system Architecture_261027_ver9/R-ECU/Actuator Control/Feedback_Sensor/Wheel Speed Feedback ==
  Bus Element In1 : Inport  PortName=Wheel_Encoder_L
  Bus Element In2 : Inport  Port=2  PortName=Wheel_Encoder_R
  Bus Element Out1 : Outport  PortName=Measured_Speed

== system Architecture_261027_ver9/R-ECU/Actuator Control/PowerTrain/Direction Control ==
  Bus Element In1 : Inport  PortName=Drive_Duty
  Bus Element In2 : Inport  Port=2  PortName=Actuator_Target
  Bus Element Out1 : Outport  PortName=Drive_Duty_Selected
  Bus Element Out2 : Outport  Port=2  PortName=Motor_Dir

== system Architecture_261027_ver9/R-ECU/Actuator Control/PowerTrain/PWM Output ==
  Bus Element In1 : Inport  PortName=Drive_Duty_Selected
  Bus Element Out1 : Outport  PortName=Motor_PWM

== system Architecture_261027_ver9/R-ECU/Actuator Control/PowerTrain/Speed Control ==
  Bus Element In1 : Inport  PortName=Target_RPM
  Bus Element In2 : Inport  Port=2  PortName=Vehicle_Feedback
  Bus Element Out1 : Outport  PortName=Drive_Duty

== system Architecture_261027_ver9/R-ECU/Actuator Control/PowerTrain/Speed Target Conversion ==
  Bus Element In1 : Inport  PortName=Actuator_Target
  Bus Element Out1 : Outport  PortName=Target_RPM

== system Architecture_261027_ver9/R-ECU/Actuator Control/Steer/Servo PWM Output ==
  Bus Element In1 : Inport  PortName=Steering_Control_Output
  Bus Element Out1 : Outport  PortName=Servo_PWM

== system Architecture_261027_ver9/R-ECU/Actuator Control/Steer/Steering Control ==
  Bus Element In1 : Inport  PortName=Steering_Error
  Bus Element Out1 : Outport  PortName=Steering_Control_Output

== system Architecture_261027_ver9/R-ECU/Actuator Control/Steer/Steering Error Calculation ==
  Bus Element In1 : Inport  PortName=Target_Steering_ADC
  Bus Element In2 : Inport  Port=2  PortName=Steer_Pot_ADC
  Bus Element Out1 : Outport  PortName=Steering_Error

== system Architecture_261027_ver9/R-ECU/Actuator Control/Steer/Steering Target Conversion ==
  Bus Element In1 : Inport  PortName=Actuator_Target
  Bus Element Out1 : Outport  PortName=Target_Steering_ADC
